simulink model "practica3ter"  (R2026b)
settings: Solver=VariableStepAuto  StopTime=10  MaxStep=0.001
libraries: fl_lib x16, nesl_utility x8, sdl_lib x2
settings Model: Creator=Ricardo Alejandro  LastModifiedBy=Ricardo Alejandro
settings SimscapeCC: SimscapeLogType=all  SimscapeNominalValues="[{\"value\":\"1\",\"unit\":\"A\"},{\"value\":\"1\",\"unit\":\"bar\"},{\"value\":\"1\",\"unit\":\"cm^2\"},{\"value\":\"1\",\"unit\":\"cm^3/s\"},{\"value\":\"1\",\"unit\":\"kJ/kg\"},{\"value\":\"1\",\"unit\":\"kW\"},{\"value\":\"1\",\"unit\":\"l\"},{\"value\":\"1\",\"unit\":\"N\"},{\"value\":\"1\",\"unit\":\"N*m\"},{\"value\":\"1\",\"unit\":\"V\"},{\"value\":\"0.001\",\"unit\":\"Wb\"}]"  SimscapeUseEnergyAccounting=off

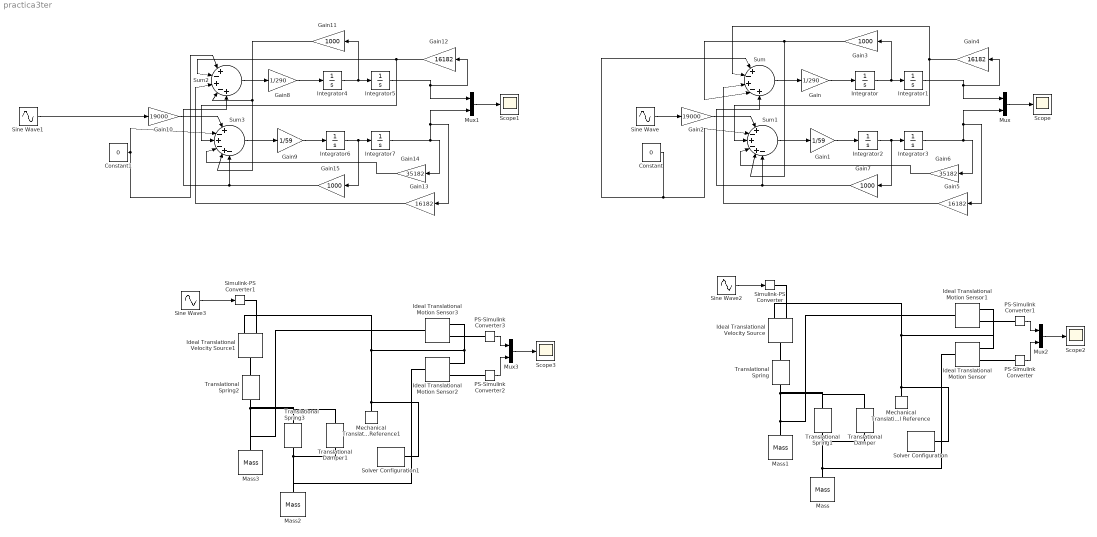
== system practica3ter ==
  Constant : Constant  Value=0
  Constant1 : Constant  Value=0
  Gain : Gain  Gain=1/290
  Gain1 : Gain  Gain=1/59
  Gain10 : Gain  Gain=19000
  Gain{3,7,11,15} (4 alike) : Gain  Gain=1000
  Gain{4..5,12..13} (4 alike) : Gain  Gain=16182
  Gain14 : Gain  Gain=35182
  Gain2 : Gain  Gain=19000
  Gain6 : Gain  Gain=35182
  Gain8 : Gain  Gain=1/290
  Gain9 : Gain  Gain=1/59
  Ideal Translational Motion Sensor{,1..3} (4 alike) : fl_lib/Mechanical/Mechanical Sensors/Ideal Translational Motion Sensor  reference=foundation.enum.MeasurementReference.difference  acceleration_port=false  velocity_port=false  position_port=true  offset=0 m
  Ideal Translational Velocity Source : fl_lib/Mechanical/Mechanical Sources/Ideal Translational Velocity Source
  Ideal Translational Velocity Source1 : fl_lib/Mechanical/Mechanical Sources/Ideal Translational Velocity Source
  Integrator{,1..7} (8 alike) : Integrator
  Mass : fl_lib/Mechanical/Translational Elements/Mass  mass=290 kg  num_ports=foundation.enum.numPorts2.one  v_specify=off  v_priority=High  v=0 m/s  v_nominal_specify=off  v_nominal_value=1  v_nominal_unit=m/s  f_specify=off  f_priority=None  f=0 N  f_nominal_specify=off  f_nominal_value=1  f_nominal_unit=N
  Mass1 : fl_lib/Mechanical/Translational Elements/Mass  mass=59 kg  num_ports=foundation.enum.numPorts2.one  v_specify=off  v_priority=High  v=0 m/s  v_nominal_specify=off  v_nominal_value=1  v_nominal_unit=m/s  f_specify=off  f_priority=None  f=0 N  f_nominal_specify=off  f_nominal_value=1  f_nominal_unit=N
  Mass2 : fl_lib/Mechanical/Translational Elements/Mass  mass=290 kg  num_ports=foundation.enum.numPorts2.one  v_specify=off  v_priority=High  v=0 m/s  v_nominal_specify=off  v_nominal_value=1  v_nominal_unit=m/s  f_specify=off  f_priority=None  f=0 N  f_nominal_specify=off  f_nominal_value=1  f_nominal_unit=N
  Mass3 : fl_lib/Mechanical/Translational Elements/Mass  mass=59 kg  num_ports=foundation.enum.numPorts2.one  v_specify=off  v_priority=High  v=0 m/s  v_nominal_specify=off  v_nominal_value=1  v_nominal_unit=m/s  f_specify=off  f_priority=None  f=0 N  f_nominal_specify=off  f_nominal_value=1  f_nominal_unit=N
  Mechanical Translational Reference : fl_lib/Mechanical/Translational Elements/Mechanical Translational Reference
  Mechanical Translational Reference1 : fl_lib/Mechanical/Translational Elements/Mechanical Translational Reference
  Mux{,1..3} (4 alike) : Mux  Inputs=2
  PS-Simulink Converter{,1..3} (4 alike) : nesl_utility/PS-Simulink Converter  PhysicalDomain=network_engine_domain  SubClassName=ps_output  LeftPortType=input  RightPortType=output  PseudoPeriodic=off  Frequencies=[]  VectorFormat=inherit  Unit=m  AffineConversion=off
  Scope{,1..3} (4 alike) : Scope
      Scope settings: ActiveDisplayYMinimum=-0.070160622724284444  ActiveDisplayYMaximum=0.080375192073623689
      Scope1 settings: ActiveDisplayYMinimum=-0.0081004107203286671  ActiveDisplayYMaximum=0.013153550265285391
      Scope2 settings: ActiveDisplayYMinimum=-0.0702507413713737  ActiveDisplayYMaximum=0.080572659109533054  DataLoggingVariableName=ScopeData2
      Scope3 settings: ActiveDisplayYMinimum=-0.008403716330010658  ActiveDisplayYMaximum=0.014221064397900189  DataLoggingVariableName=ScopeData3
  Simulink-PS Converter : nesl_utility/Simulink-PS Converter  PhysicalDomain=network_engine_domain  SubClassName=ps_input  LeftPortType=input  RightPortType=output  PseudoPeriodic=off  Frequencies=[]  NoiseDistribution=none  NoiseParameters=[]  Unit=m/s  AffineConversion=off  FilteringAndDerivatives=provide  SimscapeFilterOrder=1  InputFilterTimeConstant=0.001  UdotUserProvided=0
  Simulink-PS Converter1 : nesl_utility/Simulink-PS Converter  PhysicalDomain=network_engine_domain  SubClassName=ps_input  LeftPortType=input  RightPortType=output  PseudoPeriodic=off  Frequencies=[]  NoiseDistribution=none  NoiseParameters=[]  Unit=m/s  AffineConversion=off  FilteringAndDerivatives=provide  SimscapeFilterOrder=1  InputFilterTimeConstant=0.001  UdotUserProvided=0
  Sine Wave : Sin  Amplitude=0.05  Frequency=0.5*pi  SampleTime=0
  Sine Wave1 : Sin  Amplitude=0.05  Frequency=20*pi  SampleTime=0
  Sine Wave2 : Sin  Amplitude=0.05*0.5*pi  Frequency=0.5*pi  Phase=pi/2  SampleTime=0
  Sine Wave3 : Sin  Amplitude=0.05*20*pi  Frequency=20*pi  Phase=pi/2  SampleTime=0
  Solver Configuration : nesl_utility/Solver Configuration  PhysicalDomain=network_engine_domain  SubClassName=solver  LeftPortType=input  RightPortType=generic  Tones=[]  Harmonics=[]  SimulateNoise=off  Profile=off  UseLocalSampling=off  EnableSwitchedLinearOptims=on  FrequencyDomain=off  UseCCode=off  RelTol=0.001  AbsTol=0.001  MinStep=1e-09  ToWorkspace=off  RevertToSquareIcSolve=off  NumHomotopyIterations=100  PhasorMode=off  PhasorModeNumHarmonics=1  ConsistencySolver=NEWTON_XTOL_AFTER_FTOL  CanonicalOrdering=CANONICAL  OptimizeIntermediates=OPTIMIZED  MulticoreSolverChoice=BACKWARD_EULER  IndexReductionMethod=DerivativeReplacement  DoDC=off  ResidualTolerance=1e-09  ConsistencyTolSource=GLOBAL  ConsistencyAbsTol=0.001  ConsistencyRelTol=0.001  ConsistencyTolFactor=0.001  UseLocalSolver=off  LocalSolverChoice=NE_BACKWARD_EULER_ADVANCER  ResolveIndetEquations=on  FunctionEvalNumThread=1  LocalSolverSampleTime=0.001  DoFixedCost=off  MaxNonlinIter=3  MaxModeIter=2  ComputeImpulses=off  ImpulseIterations=2  LinearAlgebra=auto  LinearAlgebraNumThread=0  EquationFormulation=NE_TIME_EF  DelaysMemoryBudget=1024  AutomaticFiltering=on  FilteringTimeConstant=0.001  PartitionStorageMethod=AS_NEEDED  PartitionMemoryBudget=1024  PartitionMethod=BALANCED  MultibodyUseLocalSolver=off  MultibodyLocalSolverChoice=ODE1  MultibodyLocalSolverSampleTime=0.001
  Solver Configuration1 : nesl_utility/Solver Configuration  PhysicalDomain=network_engine_domain  SubClassName=solver  LeftPortType=input  RightPortType=generic  Tones=[]  Harmonics=[]  SimulateNoise=off  Profile=off  UseLocalSampling=off  EnableSwitchedLinearOptims=on  FrequencyDomain=off  UseCCode=off  RelTol=0.001  AbsTol=0.001  MinStep=1e-09  ToWorkspace=off  RevertToSquareIcSolve=off  NumHomotopyIterations=100  PhasorMode=off  PhasorModeNumHarmonics=1  ConsistencySolver=NEWTON_XTOL_AFTER_FTOL  CanonicalOrdering=CANONICAL  OptimizeIntermediates=OPTIMIZED  MulticoreSolverChoice=BACKWARD_EULER  IndexReductionMethod=DerivativeReplacement  DoDC=off  ResidualTolerance=1e-09  ConsistencyTolSource=GLOBAL  ConsistencyAbsTol=0.001  ConsistencyRelTol=0.001  ConsistencyTolFactor=0.001  UseLocalSolver=off  LocalSolverChoice=NE_BACKWARD_EULER_ADVANCER  ResolveIndetEquations=on  FunctionEvalNumThread=1  LocalSolverSampleTime=0.001  DoFixedCost=off  MaxNonlinIter=3  MaxModeIter=2  ComputeImpulses=off  ImpulseIterations=2  LinearAlgebra=auto  LinearAlgebraNumThread=0  EquationFormulation=NE_TIME_EF  DelaysMemoryBudget=1024  AutomaticFiltering=on  FilteringTimeConstant=0.001  PartitionStorageMethod=AS_NEEDED  PartitionMemoryBudget=1024  PartitionMethod=BALANCED  MultibodyUseLocalSolver=off  MultibodyLocalSolverChoice=ODE1  MultibodyLocalSolverSampleTime=0.001
  Sum : Sum  Inputs=|+-+-+
  Sum1 : Sum  Inputs=|+-+-+-
  Sum2 : Sum  Inputs=|+-+-+
  Sum3 : Sum  Inputs=|+-+-+-
  Translational Damper : sdl_lib/Couplings & Drives/Springs & Dampers/Translational Damper  D=1000 N*s/m  thermal_port=simscape.enum.thermaleffects.omit  thermal_mass=50 kJ/K  temperature_specify=off  temperature_priority=High  temperature=300 K  temperature_nominal_specify=off  temperature_nominal_value=1  temperature_nominal_unit=K
  Translational Damper1 : sdl_lib/Couplings & Drives/Springs & Dampers/Translational Damper  D=1000 N*s/m  thermal_port=simscape.enum.thermaleffects.omit  thermal_mass=50 kJ/K  temperature_specify=off  temperature_priority=High  temperature=300 K  temperature_nominal_specify=off  temperature_nominal_value=1  temperature_nominal_unit=K
  Translational Spring : fl_lib/Mechanical/Translational Elements/Translational Spring  spr_rate=19000 N/m  v_specify=off  v_priority=None  v=0 m/s  v_nominal_specify=off  v_nominal_value=1  v_nominal_unit=m/s  f_specify=off  f_priority=None  f=0 N  f_nominal_specify=off  f_nominal_value=1  f_nominal_unit=N  x_specify=off  x_priority=High  x=0 m  x_nominal_specify=off  x_nominal_value=1  x_nominal_unit=m
  Translational Spring1 : fl_lib/Mechanical/Translational Elements/Translational Spring  spr_rate=16182 N/m  v_specify=off  v_priority=None  v=0 m/s  v_nominal_specify=off  v_nominal_value=1  v_nominal_unit=m/s  f_specify=off  f_priority=None  f=0 N  f_nominal_specify=off  f_nominal_value=1  f_nominal_unit=N  x_specify=off  x_priority=High  x=0 m  x_nominal_specify=off  x_nominal_value=1  x_nominal_unit=m
  Translational Spring2 : fl_lib/Mechanical/Translational Elements/Translational Spring  spr_rate=19000 N/m  v_specify=off  v_priority=None  v=0 m/s  v_nominal_specify=off  v_nominal_value=1  v_nominal_unit=m/s  f_specify=off  f_priority=None  f=0 N  f_nominal_specify=off  f_nominal_value=1  f_nominal_unit=N  x_specify=off  x_priority=High  x=0 m  x_nominal_specify=off  x_nominal_value=1  x_nominal_unit=m
  Translational Spring3 : fl_lib/Mechanical/Translational Elements/Translational Spring  spr_rate=16182 N/m  v_specify=off  v_priority=None  v=0 m/s  v_nominal_specify=off  v_nominal_value=1  v_nominal_unit=m/s  f_specify=off  f_priority=None  f=0 N  f_nominal_specify=off  f_nominal_value=1  f_nominal_unit=N  x_specify=off  x_priority=High  x=0 m  x_nominal_specify=off  x_nominal_value=1  x_nominal_unit=m
  wires:
  Sum/1 -> Gain/1
  Sum1/1 -> Gain1/1
  Gain/1 -> Integrator/1
  Integrator/1 -> Gain3/1, Integrator1/1
  Gain1/1 -> Integrator2/1
  Integrator2/1 -> Gain7/1, Integrator3/1
  Integrator3/1 -> Gain6/1, Gain5/1, Mux/2
  Integrator1/1 -> Mux/1, Gain4/1
  Mux/1 -> Scope/1
  Sine Wave/1 -> Gain2/1
  Gain2/1 -> Sum1/1
  Constant/1 -> Sum1/2, Sum/1
  Gain4/1 -> Sum/2, Sum1/3
  Gain5/1 -> Sum/3
  Gain3/1 -> Sum1/5, Sum/4
  Gain7/1 -> Sum1/6, Sum/5
  Gain6/1 -> Sum1/4
  Gain12/1 -> Sum2/2, Sum3/3
  Integrator5/1 -> Mux1/1, Gain12/1
  Sum2/1 -> Gain8/1
  Constant1/1 -> Sum2/1, Sum3/2
  Gain9/1 -> Integrator6/1
  Gain10/1 -> Sum3/1
  Mux1/1 -> Scope1/1
  Integrator4/1 -> Gain11/1, Integrator5/1
  Integrator7/1 -> Gain14/1, Gain13/1, Mux1/2
  Gain11/1 -> Sum3/5, Sum2/4
  Integrator6/1 -> Gain15/1, Integrator7/1
  Gain13/1 -> Sum2/3
  Gain15/1 -> Sum3/6, Sum2/5
  Gain14/1 -> Sum3/4
  Sum3/1 -> Gain9/1
  Sine Wave1/1 -> Gain10/1
  Gain8/1 -> Integrator4/1
  Sine Wave2/1 -> Simulink-PS Converter/1
  Mux2/1 -> Scope2/1
  PS-Simulink Converter/1 -> Mux2/2
  PS-Simulink Converter1/1 -> Mux2/1
  Sine Wave3/1 -> Simulink-PS Converter1/1
  Mux3/1 -> Scope3/1
  PS-Simulink Converter3/1 -> Mux3/1
  PS-Simulink Converter2/1 -> Mux3/2
  connections:
  Simulink-PS Converter/RConn1 -- Ideal Translational Velocity Source/RConn1
  Translational Spring/LConn1 -- Ideal Translational Velocity Source/LConn1
  Mass1/LConn1 -- Ideal Translational Motion Sensor1/LConn1 -- Translational Damper/LConn1 -- Translational Spring1/LConn1 -- Translational Spring/RConn1
  Mass/LConn1 -- Ideal Translational Motion Sensor/LConn1 -- Translational Damper/RConn1 -- Translational Spring1/RConn1
  Ideal Translational Velocity Source/RConn2 -- Ideal Translational Motion Sensor/RConn1 -- Ideal Translational Motion Sensor1/RConn1 -- Solver Configuration/RConn1 -- Mechanical Translational Reference/LConn1
  PS-Simulink Converter/LConn1 -- Ideal Translational Motion Sensor/RConn2
  PS-Simulink Converter1/LConn1 -- Ideal Translational Motion Sensor1/RConn2
  Translational Spring2/RConn1 -- Ideal Translational Motion Sensor3/LConn1 -- Mass3/LConn1 -- Translational Damper1/LConn1 -- Translational Spring3/LConn1
  Ideal Translational Motion Sensor3/RConn1 -- Solver Configuration1/RConn1 -- Mechanical Translational Reference1/LConn1 -- Ideal Translational Velocity Source1/RConn2 -- Ideal Translational Motion Sensor2/RConn1
  Translational Spring3/RConn1 -- Ideal Translational Motion Sensor2/LConn1 -- Mass2/LConn1 -- Translational Damper1/RConn1
  Translational Spring2/LConn1 -- Ideal Translational Velocity Source1/LConn1
  Simulink-PS Converter1/RConn1 -- Ideal Translational Velocity Source1/RConn1
  PS-Simulink Converter2/LConn1 -- Ideal Translational Motion Sensor2/RConn2
  PS-Simulink Converter3/LConn1 -- Ideal Translational Motion Sensor3/RConn2
